simulink model "skarab_fgbe"  (R2018a)
settings: Solver=VariableStepDiscrete  StartTime=0.0  StopTime=50000  RelTol=1e-3
libraries: xbsIndex_r4 x704, casper_library_misc x5, xps_library x3
(part 3 of 9)

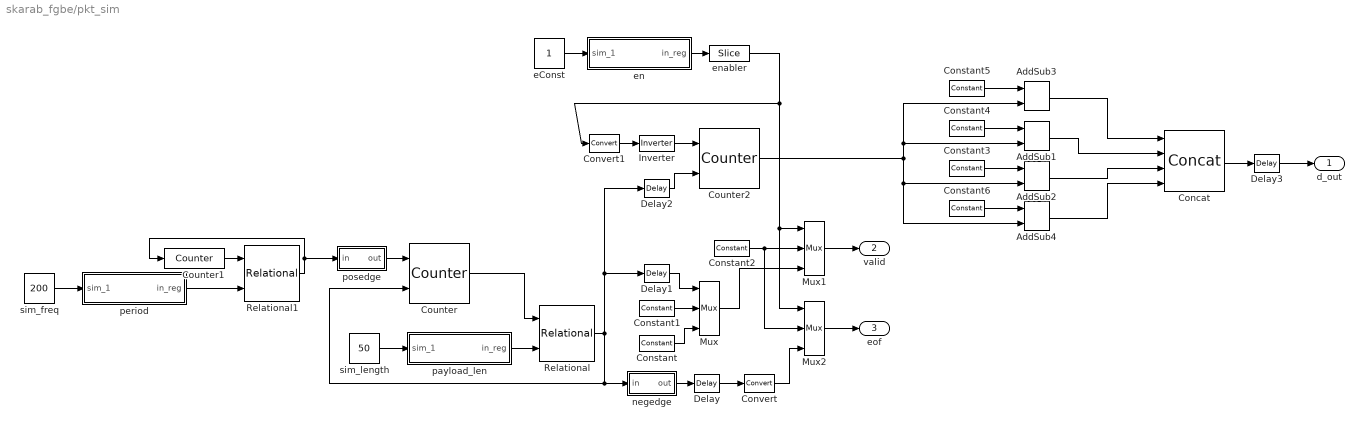
== system skarab_fgbe/pkt_sim ==
  AddSub{1..4} (4 alike) : xbsIndex_r4/AddSub  mode=Addition  use_carryin=off  use_carryout=off  en=off  latency=1  precision=User Defined  arith_type=Unsigned  n_bits=64  bin_pt=0  quantization=Truncate  overflow=Wrap  use_behavioral_HDL=off  hw_selection=Fabric  pipelined=off  dbl_ovrd=off  block_type=addsub
  Concat : xbsIndex_r4/Concat  num_inputs=4  dbl_ovrd=off  block_type=concat
  Constant : xbsIndex_r4/Constant  const=1  gui_display_data_type=Fixed-point  arith_type=Boolean  n_bits=16  bin_pt=14  preci_type=Single  exp_width=8  frac_width=24  explicit_period=on  period=1  equ=P=C  opselect=C  inp2=PCIN>>17  opr=+  inp1=P  carry=CIN  dbl_ovrd=off  block_type=constant
      settings: block_version=11.4
  Constant1 : xbsIndex_r4/Constant  const=0  gui_display_data_type=Fixed-point  arith_type=Boolean  n_bits=16  bin_pt=14  preci_type=Single  exp_width=8  frac_width=24  explicit_period=on  period=1  equ=P=C  opselect=C  inp2=PCIN>>17  opr=+  inp1=P  carry=CIN  dbl_ovrd=off  block_type=constant
      settings: block_version=11.4
  Constant2 : xbsIndex_r4/Constant  const=0  gui_display_data_type=Fixed-point  arith_type=Boolean  n_bits=16  bin_pt=14  preci_type=Single  exp_width=8  frac_width=24  explicit_period=on  period=1  equ=P=C  opselect=C  inp2=PCIN>>17  opr=+  inp1=P  carry=CIN  dbl_ovrd=off  block_type=constant
      settings: block_version=11.4
  Constant3 : xbsIndex_r4/Constant  const=3  gui_display_data_type=Fixed-point  arith_type=Unsigned  n_bits=64  bin_pt=0  preci_type=Single  exp_width=8  frac_width=24  explicit_period=off  period=1  equ=P=C  opselect=C  inp2=PCIN>>17  opr=+  inp1=P  carry=CIN  dbl_ovrd=off  block_type=constant
  Constant4 : xbsIndex_r4/Constant  const=2  gui_display_data_type=Fixed-point  arith_type=Unsigned  n_bits=64  bin_pt=0  preci_type=Single  exp_width=8  frac_width=24  explicit_period=off  period=1  equ=P=C  opselect=C  inp2=PCIN>>17  opr=+  inp1=P  carry=CIN  dbl_ovrd=off  block_type=constant
  Constant5 : xbsIndex_r4/Constant  const=1  gui_display_data_type=Fixed-point  arith_type=Unsigned  n_bits=64  bin_pt=0  preci_type=Single  exp_width=8  frac_width=24  explicit_period=off  period=1  equ=P=C  opselect=C  inp2=PCIN>>17  opr=+  inp1=P  carry=CIN  dbl_ovrd=off  block_type=constant
  Constant6 : xbsIndex_r4/Constant  const=4  gui_display_data_type=Fixed-point  arith_type=Unsigned  n_bits=64  bin_pt=0  preci_type=Single  exp_width=8  frac_width=24  explicit_period=off  period=1  equ=P=C  opselect=C  inp2=PCIN>>17  opr=+  inp1=P  carry=CIN  dbl_ovrd=off  block_type=constant
  Convert : xbsIndex_r4/Convert  gui_display_data_type=Fixed-point  arith_type=Boolean  n_bits=16  bin_pt=14  float_type=Single  exp_bits=8  fraction_bits=24  quantization=Truncate  overflow=Wrap  en=off  latency=0  pipeline=off  dbl_ovrd=off  block_type=convert
      settings: block_version=11.4
  Convert1 : xbsIndex_r4/Convert  gui_display_data_type=Fixed-point  arith_type=Boolean  n_bits=16  bin_pt=14  float_type=Single  exp_bits=8  fraction_bits=24  quantization=Truncate  overflow=Wrap  en=off  latency=0  pipeline=off  dbl_ovrd=off  block_type=convert
      settings: block_version=11.4
  Counter : xbsIndex_r4/Counter  cnt_type=Free Running  cnt_to=Inf  operation=Up  start_count=0  cnt_by_val=1  arith_type=Unsigned  n_bits=32  bin_pt=0  load_pin=off  rst=on  en=on  explicit_period=on  period=1  use_behavioral_HDL=off  implementation=Fabric  dbl_ovrd=off  block_type=counter
      settings: block_version=11.4
  Counter1 : xbsIndex_r4/Counter  cnt_type=Free Running  cnt_to=Inf  operation=Up  start_count=1  cnt_by_val=1  arith_type=Unsigned  n_bits=32  bin_pt=0  load_pin=off  rst=on  en=off  explicit_period=on  period=1  use_behavioral_HDL=off  implementation=Fabric  dbl_ovrd=off  block_type=counter
      settings: block_version=11.4
  Counter2 : xbsIndex_r4/Counter  cnt_type=Free Running  cnt_to=Inf  operation=Up  start_count=0  cnt_by_val=1  arith_type=Unsigned  n_bits=64  bin_pt=0  load_pin=off  rst=on  en=on  explicit_period=off  period=1  use_behavioral_HDL=off  implementation=Fabric  dbl_ovrd=off  block_type=counter
      settings: block_version=11.4
  Delay{,1..3} (4 alike) : xbsIndex_r4/Delay  rst=off  infoeditControl=Selection of Reset will increase slice count due to use of real FFs and instead of SRLs  en=off  latency=1  reg_retiming=on  dbl_ovrd=off  block_type=delay
      settings: block_version=11.4
  Inverter : xbsIndex_r4/Inverter  en=off  latency=0  dbl_ovrd=off  block_type=inv
      settings: block_version=11.4
  Mux : xbsIndex_r4/Mux  inputs=2  en=off  latency=1  precision=Full  arith_type=Unsigned  n_bits=16  bin_pt=14  quantization=Truncate  overflow=Wrap  dbl_ovrd=off  block_type=mux
      settings: block_version=11.4
  Mux1 : xbsIndex_r4/Mux  inputs=2  en=off  latency=1  precision=Full  arith_type=Unsigned  n_bits=16  bin_pt=14  quantization=Truncate  overflow=Wrap  dbl_ovrd=off  block_type=mux
      settings: block_version=11.4
  Mux2 : xbsIndex_r4/Mux  inputs=2  en=off  latency=1  precision=Full  arith_type=Unsigned  n_bits=16  bin_pt=14  quantization=Truncate  overflow=Wrap  dbl_ovrd=off  block_type=mux
      settings: block_version=11.4
  Relational : xbsIndex_r4/Relational  mode=a<b  op_type=Bool  en=off  latency=0  dbl_ovrd=off  block_type=relational
  Relational1 : xbsIndex_r4/Relational  mode=a>=b  op_type=Bool  en=off  latency=0  dbl_ovrd=off  block_type=relational
  eConst : Constant
  en : Subsystem  Tag=xps:sw_reg  AncestorBlock=xps_library/Memory/software_register  mask(swreg){io_dir=From Processor, io_delay=0, init_val=234000, sample_period=1, names=reg, bitwidths=32, bin_pts=0, arith_types=0, sim_port=on, show_format=on}
      mask prompts: io_dir "I/O direction"; io_delay "I/O delay"; init_val "Initial Value"; sample_period "Sample period"; names "Bitfield names [msb...lsb]"; bitwidths "Bitfield widths"; bin_pts "Bitfield binary pts"; arith_types "Bitfield types, ufix=0, fix=1, bool=2"; sim_port "Provide sim input/output?"; show_format "Print format string?"
      mask help: A 32-bit software-accessible register. Can be divided into bitfields of varying widths and types using the fields in the block mask.
      mask init:
      | swreg_init(gcb)
      settings: AttributesFormatString=1input:uf32.0 = 32 bits
      mask TypeOptions io_dir: To Processor | From Processor
      mask Callback io_dir:
      | mask_enables = get_param(gcb, 'MaskEnables');
      | mask_names = get_param(gcb, 'MaskNames');
      | if strcmp(get_param(gcb, 'io_dir'), 'To Processor'),
      |     mask_enables{ismember(mask_names, 'sample_period')} = 'off';
      | else
      |     mask_enables{ismember(mask_names, 'sample_period')} = 'on';
      | end
      | set_param(gcb, 'MaskEnables', mask_enables);
      mask DialogControl ParameterTabVar0 Prompt: Setup
  enabler : xbsIndex_r4/Slice  nbits=1  boolean_output=off  mode=Lower Bit Location + Width  bit1=0  base1=MSB of Input  bit0=0  base0=LSB of Input  dbl_ovrd=off  block_type=slice
  negedge : Subsystem  AncestorBlock=casper_library_misc/edge_detect  mask(edge_detect){edge=Falling, polarity=Active High, x_in=[0 0.08 0.08 0.16 0.16 0.24 0.24 0.32 0.32 0.4], y_in=[-1 -1  1  1  1  1  1  1  1  1], x_out=[0.6 0.68 0.68 0.76 0.76 0.84 0.84 0.92 0.92 1], y_out=[-1 -1  1  1 -1 -1 -1 -1 -1 -1]}
      mask prompts: edge "Edge Type"; polarity "Output Polarity"; x_in "Input X Positions"; y_in "Input Y Positions"; x_out "Output X Positions"; y_out "Output Y Positions"
      mask help: Output is active for one-cycle after each edge of the specified type (i.e. rising, falling or both).
      mask init:
      | edge_detect_init(gcb,...
      |     'edge',edge,...
      |     'polarity',polarity,...
      |     'x_in',x_in,...
      |     'x_out',x_out,...
      |     'y_in',y_in,...
      |     'y_out',y_out);
      | 
      | x_in_num=str2num(getfield(getfield(get_param(gcb,'UserData'),'parameters'),'x_in'));
      | x_out_num=str2num(getfield(getfield(get_param(gcb,'UserData'),'parameters'),'x_out'));
      | y_in_num=str2num(getfield(getfield(get_param(gcb,'UserData'),'parameters'),'y_in'));
      | y_out_num=str2num(getfield(getfield(get_param(gcb,'UserData'),'parameters'),'y_out'));
      settings: AttributesFormatString=|
      | falling edges
      | active high
      mask Help: Output is active for one-cycle after each edge of the specified type (i.e. rising, falling, or both).  Latency is zero.
      mask TypeOptions edge: Rising | Falling | Both
      mask TypeOptions polarity: Active High | Active Low
      mask Display:
      | plot(x_in_num,0.5+y_in_num*0.2);
      | plot(x_out_num,0.5+y_out_num*0.2);
  payload_len : Subsystem  Tag=xps:sw_reg  AncestorBlock=xps_library/Memory/software_register  mask(swreg){io_dir=From Processor, io_delay=0, init_val=654, sample_period=1, names=reg, bitwidths=32, bin_pts=0, arith_types=0, sim_port=on, show_format=on}
      mask prompts: io_dir "I/O direction"; io_delay "I/O delay"; init_val "Initial Value"; sample_period "Sample period"; names "Bitfield names [msb...lsb]"; bitwidths "Bitfield widths"; bin_pts "Bitfield binary pts"; arith_types "Bitfield types, ufix=0, fix=1, bool=2"; sim_port "Provide sim input/output?"; show_format "Print format string?"
      mask help: A 32-bit software-accessible register. Can be divided into bitfields of varying widths and types using the fields in the block mask.
      mask init:
      | swreg_init(gcb)
      settings: AttributesFormatString=1input:uf32.0 = 32 bits
      mask TypeOptions io_dir: To Processor | From Processor
      mask Callback io_dir:
      | mask_enables = get_param(gcb, 'MaskEnables');
      | mask_names = get_param(gcb, 'MaskNames');
      | if strcmp(get_param(gcb, 'io_dir'), 'To Processor'),
      |     mask_enables{ismember(mask_names, 'sample_period')} = 'off';
      | else
      |     mask_enables{ismember(mask_names, 'sample_period')} = 'on';
      | end
      | set_param(gcb, 'MaskEnables', mask_enables);
      mask DialogControl ParameterTabVar0 Prompt: Setup
  period : Subsystem  Tag=xps:sw_reg  AncestorBlock=xps_library/Memory/software_register  mask(swreg){io_dir=From Processor, io_delay=0, init_val=1000, sample_period=1, names=reg, bitwidths=32, bin_pts=0, arith_types=0, sim_port=on, show_format=on}
      mask prompts: io_dir "I/O direction"; io_delay "I/O delay"; init_val "Initial Value"; sample_period "Sample period"; names "Bitfield names [msb...lsb]"; bitwidths "Bitfield widths"; bin_pts "Bitfield binary pts"; arith_types "Bitfield types, ufix=0, fix=1, bool=2"; sim_port "Provide sim input/output?"; show_format "Print format string?"
      mask help: A 32-bit software-accessible register. Can be divided into bitfields of varying widths and types using the fields in the block mask.
      mask init:
      | swreg_init(gcb)
      settings: AttributesFormatString=1input:uf32.0 = 32 bits
      mask TypeOptions io_dir: To Processor | From Processor
      mask Callback io_dir:
      | mask_enables = get_param(gcb, 'MaskEnables');
      | mask_names = get_param(gcb, 'MaskNames');
      | if strcmp(get_param(gcb, 'io_dir'), 'To Processor'),
      |     mask_enables{ismember(mask_names, 'sample_period')} = 'off';
      | else
      |     mask_enables{ismember(mask_names, 'sample_period')} = 'on';
      | end
      | set_param(gcb, 'MaskEnables', mask_enables);
      mask DialogControl ParameterTabVar0 Prompt: Setup
  posedge : Subsystem  AncestorBlock=casper_library_misc/edge_detect  mask(edge_detect){edge=Rising, polarity=Active High, x_in=[0 0.08 0.08 0.16 0.16 0.24 0.24 0.32 0.32 0.4], y_in=[-1 -1  1  1  1  1  1  1  1  1], x_out=[0.6 0.68 0.68 0.76 0.76 0.84 0.84 0.92 0.92 1], y_out=[-1 -1  1  1 -1 -1 -1 -1 -1 -1]}
      mask prompts: edge "Edge Type"; polarity "Output Polarity"; x_in "Input X Positions"; y_in "Input Y Positions"; x_out "Output X Positions"; y_out "Output Y Positions"
      mask help: Output is active for one-cycle after each edge of the specified type (i.e. rising, falling or both).
      mask init: same as skarab_fgbe/pkt_sim/negedge
      settings: AttributesFormatString=|
      | rising edges
      | active high
      mask Help: Output is active for one-cycle after each edge of the specified type (i.e. rising, falling, or both).  Latency is zero.
      mask TypeOptions edge: Rising | Falling | Both
      mask TypeOptions polarity: Active High | Active Low
      mask Display:
      | plot(x_in_num,0.5+y_in_num*0.2);
      | plot(x_out_num,0.5+y_out_num*0.2);
  sim_freq : Constant  Value=200
  sim_length : Constant  Value=50
  d_out : Outport
  valid : Outport  Port=2
  eof : Outport  Port=3
  wires:
  Counter/1 -> Relational/1
  sim_length/1 -> payload_len/1(sim_1)
  posedge/1(out) -> Counter/1
  Mux2/1 -> eof/1
  Mux1/1 -> valid/1
  Delay3/1 -> d_out/1
  enabler/1 -> Mux1/1, Mux2/1, Convert1/1
  en/1(in_reg) -> enabler/1
  eConst/1 -> en/1(sim_1)
  Convert1/1 -> Inverter/1
  Inverter/1 -> Counter2/1
  Delay2/1 -> Counter2/2
  Convert/1 -> Mux2/3
  Constant2/1 -> Mux1/2, Mux2/2
  Mux/1 -> Mux1/3
  Delay1/1 -> Mux/1
  Constant/1 -> Mux/3
  Constant1/1 -> Mux/2
  Delay/1 -> Convert/1
  negedge/1(out) -> Delay/1
  Relational1/1 -> posedge/1(in), Counter1/1
  Counter1/1 -> Relational1/1
  period/1(in_reg) -> Relational1/2
  sim_freq/1 -> period/1(sim_1)
  Relational/1 -> negedge/1(in), Counter/2, Delay1/1, Delay2/1
  payload_len/1(in_reg) -> Relational/2
  Constant5/1 -> AddSub3/1
  Constant4/1 -> AddSub1/1
  Constant3/1 -> AddSub2/1
  Constant6/1 -> AddSub4/1
  Counter2/1 -> AddSub1/2, AddSub3/2, AddSub2/2, AddSub4/2
  AddSub3/1 -> Concat/1
  AddSub1/1 -> Concat/2
  AddSub2/1 -> Concat/3
  AddSub4/1 -> Concat/4
  Concat/1 -> Delay3/1

== system skarab_fgbe/rst ==
  sim_1 : Inport
  convert1_1 : DataTypeConversion  OutDataTypeStr=fixdt('ufix32_En0')  LockScale=on
  convert2_1 : DataTypeConversion  OutDataTypeStr=fixdt('ufix32_En0')  ConvertRealWorld=Stored Integer (SI)  LockScale=on
  gain_1 : Gain
  io_delay : xbsIndex_r4/Delay  rst=off  infoeditControl=Selection of Reset will increase slice count due to use of real FFs and instead of SRLs  en=off  latency=0  reg_retiming=on  dbl_ovrd=off  block_type=delay
  reint1 : xbsIndex_r4/Reinterpret  force_arith_type=on  arith_type=Unsigned  force_bin_pt=on  bin_pt=0  block_type=reinterpret
  skarab_fgbe_rst_user_data_out : xbsIndex_r4/Gateway In  gui_display_data_type=Fixed-point  arith_type=Unsigned  n_bits=32  bin_pt=0  preci_type=Single  exp_width=8  frac_width=24  rows=1  columns=1  quantization="Round  (unbiased: +/- Inf)"  overflow=Saturate  period=1  UseAsADC=off  ADCChannel='1'  interface=None  automatic_assignment=on  address_offset=hex2dec('00')  intf_name=''  intf_description=''  default_value=0  timing_constraint=None  locs_specified=off  LOCs={}  io_standard={}  inherit_from_input=off  hdl_port=on  dbl_ovrd=off  block_type=gatewayin
  slice_reg : xbsIndex_r4/Slice  nbits=32  boolean_output=off  mode=Lower Bit Location + Width  bit1=0  base1=MSB of Input  bit0=0  base0=LSB of Input  dbl_ovrd=off  block_type=slice
  in_reg : Outport
  wires:
  skarab_fgbe_rst_user_data_out/1 -> io_delay/1
  sim_1/1 -> convert1_1/1
  convert1_1/1 -> convert2_1/1
  convert2_1/1 -> gain_1/1
  gain_1/1 -> skarab_fgbe_rst_user_data_out/1
  io_delay/1 -> slice_reg/1
  slice_reg/1 -> reint1/1
  reint1/1 -> in_reg/1

== system skarab_fgbe/rx ==
  out_reg : Inport
  assert_reg : xbsIndex_r4/Assert  assert_type=on  type_source=Explicitly  gui_display_data_type=Fixed-point  arith_type=Unsigned  n_bits=32  bin_pt=0  preci_type=Single  exp_width=8  frac_width=24  assert_rate=off  rate_source=Explicitly  period=1  output_port=on  block_type=assert
  cast_gw : xbsIndex_r4/Convert  gui_display_data_type=Fixed-point  arith_type=Unsigned  n_bits=32  bin_pt=0  float_type=Single  exp_bits=8  fraction_bits=24  quantization=Truncate  overflow=Wrap  en=off  latency=1  pipeline=off  dbl_ovrd=off  block_type=convert
  io_delay : xbsIndex_r4/Delay  rst=off  infoeditControl=Selection of Reset will increase slice count due to use of real FFs and instead of SRLs  en=off  latency=0  reg_retiming=on  dbl_ovrd=off  block_type=delay
  reint1 : xbsIndex_r4/Reinterpret  force_arith_type=on  arith_type=Unsigned  force_bin_pt=on  bin_pt=0  block_type=reinterpret
  sim_out : Terminator
  sim_out_reg_gw : xbsIndex_r4/Gateway Out  inherit_from_input=off  hdl_port=off  rows=1  columns=1  UseAsDAC=off  DACChannel='1'  interface=None  automatic_assignment=on  address_offset=hex2dec('00')  intf_name=''  intf_description=''  timing_constraint=None  locs_specified=off  LOCs={}  io_standard={}  block_type=gatewayout
  sim_out_reg_sim_delay : xbsIndex_r4/Delay  rst=off  infoeditControl=Selection of Reset will increase slice count due to use of real FFs and instead of SRLs  en=off  latency=1  reg_retiming=on  dbl_ovrd=off  block_type=delay
  skarab_fgbe_rx_user_data_in : xbsIndex_r4/Gateway Out  inherit_from_input=off  hdl_port=on  rows=1  columns=1  UseAsDAC=off  DACChannel='1'  interface=None  automatic_assignment=on  address_offset=hex2dec('00')  intf_name=''  intf_description=''  timing_constraint=None  locs_specified=off  LOCs={}  io_standard={}  block_type=gatewayout
  sim_out_reg : Outport
  wires:
  sim_out_reg_sim_delay/1 -> sim_out_reg_gw/1
  sim_out_reg_gw/1 -> sim_out_reg/1
  io_delay/1 -> cast_gw/1
  cast_gw/1 -> skarab_fgbe_rx_user_data_in/1
  skarab_fgbe_rx_user_data_in/1 -> sim_out/1
  out_reg/1 -> sim_out_reg_sim_delay/1, assert_reg/1
  assert_reg/1 -> reint1/1
  reint1/1 -> io_delay/1

== system skarab_fgbe/rx_bad_frame ==
  out_reg : Inport
  assert_reg : xbsIndex_r4/Assert  assert_type=on  type_source=Explicitly  gui_display_data_type=Fixed-point  arith_type=Unsigned  n_bits=32  bin_pt=0  preci_type=Single  exp_width=8  frac_width=24  assert_rate=off  rate_source=Explicitly  period=1  output_port=on  block_type=assert
  cast_gw : xbsIndex_r4/Convert  gui_display_data_type=Fixed-point  arith_type=Unsigned  n_bits=32  bin_pt=0  float_type=Single  exp_bits=8  fraction_bits=24  quantization=Truncate  overflow=Wrap  en=off  latency=1  pipeline=off  dbl_ovrd=off  block_type=convert
  io_delay : xbsIndex_r4/Delay  rst=off  infoeditControl=Selection of Reset will increase slice count due to use of real FFs and instead of SRLs  en=off  latency=0  reg_retiming=on  dbl_ovrd=off  block_type=delay
  reint1 : xbsIndex_r4/Reinterpret  force_arith_type=on  arith_type=Unsigned  force_bin_pt=on  bin_pt=0  block_type=reinterpret
  sim_out : Terminator
  sim_out_reg_gw : xbsIndex_r4/Gateway Out  inherit_from_input=off  hdl_port=off  rows=1  columns=1  UseAsDAC=off  DACChannel='1'  interface=None  automatic_assignment=on  address_offset=hex2dec('00')  intf_name=''  intf_description=''  timing_constraint=None  locs_specified=off  LOCs={}  io_standard={}  block_type=gatewayout
  sim_out_reg_sim_delay : xbsIndex_r4/Delay  rst=off  infoeditControl=Selection of Reset will increase slice count due to use of real FFs and instead of SRLs  en=off  latency=1  reg_retiming=on  dbl_ovrd=off  block_type=delay
  skarab_fgbe_rx_bad_frame_user_data_in : xbsIndex_r4/Gateway Out  inherit_from_input=off  hdl_port=on  rows=1  columns=1  UseAsDAC=off  DACChannel='1'  interface=None  automatic_assignment=on  address_offset=hex2dec('00')  intf_name=''  intf_description=''  timing_constraint=None  locs_specified=off  LOCs={}  io_standard={}  block_type=gatewayout
  sim_out_reg : Outport
  wires:
  sim_out_reg_sim_delay/1 -> sim_out_reg_gw/1
  sim_out_reg_gw/1 -> sim_out_reg/1
  io_delay/1 -> cast_gw/1
  cast_gw/1 -> skarab_fgbe_rx_bad_frame_user_data_in/1
  skarab_fgbe_rx_bad_frame_user_data_in/1 -> sim_out/1
  out_reg/1 -> sim_out_reg_sim_delay/1, assert_reg/1
  assert_reg/1 -> reint1/1
  reint1/1 -> io_delay/1

== system skarab_fgbe/rx_data ==
  out_reg : Inport
  assert_reg : xbsIndex_r4/Assert  assert_type=on  type_source=Explicitly  gui_display_data_type=Fixed-point  arith_type=Unsigned  n_bits=32  bin_pt=0  preci_type=Single  exp_width=8  frac_width=24  assert_rate=off  rate_source=Explicitly  period=1  output_port=on  block_type=assert
  cast_gw : xbsIndex_r4/Convert  gui_display_data_type=Fixed-point  arith_type=Unsigned  n_bits=32  bin_pt=0  float_type=Single  exp_bits=8  fraction_bits=24  quantization=Truncate  overflow=Wrap  en=off  latency=1  pipeline=off  dbl_ovrd=off  block_type=convert
  io_delay : xbsIndex_r4/Delay  rst=off  infoeditControl=Selection of Reset will increase slice count due to use of real FFs and instead of SRLs  en=off  latency=0  reg_retiming=on  dbl_ovrd=off  block_type=delay
  reint1 : xbsIndex_r4/Reinterpret  force_arith_type=on  arith_type=Unsigned  force_bin_pt=on  bin_pt=0  block_type=reinterpret
  sim_out : Terminator
  sim_out_reg_gw : xbsIndex_r4/Gateway Out  inherit_from_input=off  hdl_port=off  rows=1  columns=1  UseAsDAC=off  DACChannel='1'  interface=None  automatic_assignment=on  address_offset=hex2dec('00')  intf_name=''  intf_description=''  timing_constraint=None  locs_specified=off  LOCs={}  io_standard={}  block_type=gatewayout
  sim_out_reg_sim_delay : xbsIndex_r4/Delay  rst=off  infoeditControl=Selection of Reset will increase slice count due to use of real FFs and instead of SRLs  en=off  latency=1  reg_retiming=on  dbl_ovrd=off  block_type=delay
  skarab_fgbe_rx_data_user_data_in : xbsIndex_r4/Gateway Out  inherit_from_input=off  hdl_port=on  rows=1  columns=1  UseAsDAC=off  DACChannel='1'  interface=None  automatic_assignment=on  address_offset=hex2dec('00')  intf_name=''  intf_description=''  timing_constraint=None  locs_specified=off  LOCs={}  io_standard={}  block_type=gatewayout
  sim_out_reg : Outport
  wires:
  sim_out_reg_sim_delay/1 -> sim_out_reg_gw/1
  sim_out_reg_gw/1 -> sim_out_reg/1
  io_delay/1 -> cast_gw/1
  cast_gw/1 -> skarab_fgbe_rx_data_user_data_in/1
  skarab_fgbe_rx_data_user_data_in/1 -> sim_out/1
  out_reg/1 -> sim_out_reg_sim_delay/1, assert_reg/1
  assert_reg/1 -> reint1/1
  reint1/1 -> io_delay/1

== system skarab_fgbe/rx_dest_ip ==
  out_reg : Inport
  assert_reg : xbsIndex_r4/Assert  assert_type=on  type_source=Explicitly  gui_display_data_type=Fixed-point  arith_type=Unsigned  n_bits=32  bin_pt=0  preci_type=Single  exp_width=8  frac_width=24  assert_rate=off  rate_source=Explicitly  period=1  output_port=on  block_type=assert
  cast_gw : xbsIndex_r4/Convert  gui_display_data_type=Fixed-point  arith_type=Unsigned  n_bits=32  bin_pt=0  float_type=Single  exp_bits=8  fraction_bits=24  quantization=Truncate  overflow=Wrap  en=off  latency=1  pipeline=off  dbl_ovrd=off  block_type=convert
  io_delay : xbsIndex_r4/Delay  rst=off  infoeditControl=Selection of Reset will increase slice count due to use of real FFs and instead of SRLs  en=off  latency=0  reg_retiming=on  dbl_ovrd=off  block_type=delay
  reint1 : xbsIndex_r4/Reinterpret  force_arith_type=on  arith_type=Unsigned  force_bin_pt=on  bin_pt=0  block_type=reinterpret
  sim_out : Terminator
  sim_out_reg_gw : xbsIndex_r4/Gateway Out  inherit_from_input=off  hdl_port=off  rows=1  columns=1  UseAsDAC=off  DACChannel='1'  interface=None  automatic_assignment=on  address_offset=hex2dec('00')  intf_name=''  intf_description=''  timing_constraint=None  locs_specified=off  LOCs={}  io_standard={}  block_type=gatewayout
  sim_out_reg_sim_delay : xbsIndex_r4/Delay  rst=off  infoeditControl=Selection of Reset will increase slice count due to use of real FFs and instead of SRLs  en=off  latency=1  reg_retiming=on  dbl_ovrd=off  block_type=delay
  skarab_fgbe_rx_dest_ip_user_data_in : xbsIndex_r4/Gateway Out  inherit_from_input=off  hdl_port=on  rows=1  columns=1  UseAsDAC=off  DACChannel='1'  interface=None  automatic_assignment=on  address_offset=hex2dec('00')  intf_name=''  intf_description=''  timing_constraint=None  locs_specified=off  LOCs={}  io_standard={}  block_type=gatewayout
  sim_out_reg : Outport
  wires:
  sim_out_reg_sim_delay/1 -> sim_out_reg_gw/1
  sim_out_reg_gw/1 -> sim_out_reg/1
  io_delay/1 -> cast_gw/1
  cast_gw/1 -> skarab_fgbe_rx_dest_ip_user_data_in/1
  skarab_fgbe_rx_dest_ip_user_data_in/1 -> sim_out/1
  out_reg/1 -> sim_out_reg_sim_delay/1, assert_reg/1
  assert_reg/1 -> reint1/1
  reint1/1 -> io_delay/1

== system skarab_fgbe/rx_dest_port ==
  out_reg : Inport
  assert_reg : xbsIndex_r4/Assert  assert_type=on  type_source=Explicitly  gui_display_data_type=Fixed-point  arith_type=Unsigned  n_bits=32  bin_pt=0  preci_type=Single  exp_width=8  frac_width=24  assert_rate=off  rate_source=Explicitly  period=1  output_port=on  block_type=assert
  cast_gw : xbsIndex_r4/Convert  gui_display_data_type=Fixed-point  arith_type=Unsigned  n_bits=32  bin_pt=0  float_type=Single  exp_bits=8  fraction_bits=24  quantization=Truncate  overflow=Wrap  en=off  latency=1  pipeline=off  dbl_ovrd=off  block_type=convert
  io_delay : xbsIndex_r4/Delay  rst=off  infoeditControl=Selection of Reset will increase slice count due to use of real FFs and instead of SRLs  en=off  latency=0  reg_retiming=on  dbl_ovrd=off  block_type=delay
  reint1 : xbsIndex_r4/Reinterpret  force_arith_type=on  arith_type=Unsigned  force_bin_pt=on  bin_pt=0  block_type=reinterpret
  sim_out : Terminator
  sim_out_reg_gw : xbsIndex_r4/Gateway Out  inherit_from_input=off  hdl_port=off  rows=1  columns=1  UseAsDAC=off  DACChannel='1'  interface=None  automatic_assignment=on  address_offset=hex2dec('00')  intf_name=''  intf_description=''  timing_constraint=None  locs_specified=off  LOCs={}  io_standard={}  block_type=gatewayout
  sim_out_reg_sim_delay : xbsIndex_r4/Delay  rst=off  infoeditControl=Selection of Reset will increase slice count due to use of real FFs and instead of SRLs  en=off  latency=1  reg_retiming=on  dbl_ovrd=off  block_type=delay
  skarab_fgbe_rx_dest_port_user_data_in : xbsIndex_r4/Gateway Out  inherit_from_input=off  hdl_port=on  rows=1  columns=1  UseAsDAC=off  DACChannel='1'  interface=None  automatic_assignment=on  address_offset=hex2dec('00')  intf_name=''  intf_description=''  timing_constraint=None  locs_specified=off  LOCs={}  io_standard={}  block_type=gatewayout
  sim_out_reg : Outport
  wires:
  sim_out_reg_sim_delay/1 -> sim_out_reg_gw/1
  sim_out_reg_gw/1 -> sim_out_reg/1
  io_delay/1 -> cast_gw/1
  cast_gw/1 -> skarab_fgbe_rx_dest_port_user_data_in/1
  skarab_fgbe_rx_dest_port_user_data_in/1 -> sim_out/1
  out_reg/1 -> sim_out_reg_sim_delay/1, assert_reg/1
  assert_reg/1 -> reint1/1
  reint1/1 -> io_delay/1

== system skarab_fgbe/rx_end_of_frame ==
  out_reg : Inport
  assert_reg : xbsIndex_r4/Assert  assert_type=on  type_source=Explicitly  gui_display_data_type=Fixed-point  arith_type=Unsigned  n_bits=32  bin_pt=0  preci_type=Single  exp_width=8  frac_width=24  assert_rate=off  rate_source=Explicitly  period=1  output_port=on  block_type=assert
  cast_gw : xbsIndex_r4/Convert  gui_display_data_type=Fixed-point  arith_type=Unsigned  n_bits=32  bin_pt=0  float_type=Single  exp_bits=8  fraction_bits=24  quantization=Truncate  overflow=Wrap  en=off  latency=1  pipeline=off  dbl_ovrd=off  block_type=convert
  io_delay : xbsIndex_r4/Delay  rst=off  infoeditControl=Selection of Reset will increase slice count due to use of real FFs and instead of SRLs  en=off  latency=0  reg_retiming=on  dbl_ovrd=off  block_type=delay
  reint1 : xbsIndex_r4/Reinterpret  force_arith_type=on  arith_type=Unsigned  force_bin_pt=on  bin_pt=0  block_type=reinterpret
  sim_out : Terminator
  sim_out_reg_gw : xbsIndex_r4/Gateway Out  inherit_from_input=off  hdl_port=off  rows=1  columns=1  UseAsDAC=off  DACChannel='1'  interface=None  automatic_assignment=on  address_offset=hex2dec('00')  intf_name=''  intf_description=''  timing_constraint=None  locs_specified=off  LOCs={}  io_standard={}  block_type=gatewayout
  sim_out_reg_sim_delay : xbsIndex_r4/Delay  rst=off  infoeditControl=Selection of Reset will increase slice count due to use of real FFs and instead of SRLs  en=off  latency=1  reg_retiming=on  dbl_ovrd=off  block_type=delay
  skarab_fgbe_rx_end_of_frame_user_data_in : xbsIndex_r4/Gateway Out  inherit_from_input=off  hdl_port=on  rows=1  columns=1  UseAsDAC=off  DACChannel='1'  interface=None  automatic_assignment=on  address_offset=hex2dec('00')  intf_name=''  intf_description=''  timing_constraint=None  locs_specified=off  LOCs={}  io_standard={}  block_type=gatewayout
  sim_out_reg : Outport
  wires:
  sim_out_reg_sim_delay/1 -> sim_out_reg_gw/1
  sim_out_reg_gw/1 -> sim_out_reg/1
  io_delay/1 -> cast_gw/1
  cast_gw/1 -> skarab_fgbe_rx_end_of_frame_user_data_in/1
  skarab_fgbe_rx_end_of_frame_user_data_in/1 -> sim_out/1
  out_reg/1 -> sim_out_reg_sim_delay/1, assert_reg/1
  assert_reg/1 -> reint1/1
  reint1/1 -> io_delay/1

== system skarab_fgbe/rx_valid ==
  out_reg : Inport
  assert_reg : xbsIndex_r4/Assert  assert_type=on  type_source=Explicitly  gui_display_data_type=Fixed-point  arith_type=Unsigned  n_bits=32  bin_pt=0  preci_type=Single  exp_width=8  frac_width=24  assert_rate=off  rate_source=Explicitly  period=1  output_port=on  block_type=assert
  cast_gw : xbsIndex_r4/Convert  gui_display_data_type=Fixed-point  arith_type=Unsigned  n_bits=32  bin_pt=0  float_type=Single  exp_bits=8  fraction_bits=24  quantization=Truncate  overflow=Wrap  en=off  latency=1  pipeline=off  dbl_ovrd=off  block_type=convert
  io_delay : xbsIndex_r4/Delay  rst=off  infoeditControl=Selection of Reset will increase slice count due to use of real FFs and instead of SRLs  en=off  latency=0  reg_retiming=on  dbl_ovrd=off  block_type=delay
  reint1 : xbsIndex_r4/Reinterpret  force_arith_type=on  arith_type=Unsigned  force_bin_pt=on  bin_pt=0  block_type=reinterpret
  sim_out : Terminator
  sim_out_reg_gw : xbsIndex_r4/Gateway Out  inherit_from_input=off  hdl_port=off  rows=1  columns=1  UseAsDAC=off  DACChannel='1'  interface=None  automatic_assignment=on  address_offset=hex2dec('00')  intf_name=''  intf_description=''  timing_constraint=None  locs_specified=off  LOCs={}  io_standard={}  block_type=gatewayout
  sim_out_reg_sim_delay : xbsIndex_r4/Delay  rst=off  infoeditControl=Selection of Reset will increase slice count due to use of real FFs and instead of SRLs  en=off  latency=1  reg_retiming=on  dbl_ovrd=off  block_type=delay
  skarab_fgbe_rx_valid_user_data_in : xbsIndex_r4/Gateway Out  inherit_from_input=off  hdl_port=on  rows=1  columns=1  UseAsDAC=off  DACChannel='1'  interface=None  automatic_assignment=on  address_offset=hex2dec('00')  intf_name=''  intf_description=''  timing_constraint=None  locs_specified=off  LOCs={}  io_standard={}  block_type=gatewayout
  sim_out_reg : Outport
  wires:
  sim_out_reg_sim_delay/1 -> sim_out_reg_gw/1
  sim_out_reg_gw/1 -> sim_out_reg/1
  io_delay/1 -> cast_gw/1
  cast_gw/1 -> skarab_fgbe_rx_valid_user_data_in/1
  skarab_fgbe_rx_valid_user_data_in/1 -> sim_out/1
  out_reg/1 -> sim_out_reg_sim_delay/1, assert_reg/1
  assert_reg/1 -> reint1/1
  reint1/1 -> io_delay/1

== system skarab_fgbe/tx ==
  out_reg : Inport
  assert_reg : xbsIndex_r4/Assert  assert_type=on  type_source=Explicitly  gui_display_data_type=Fixed-point  arith_type=Unsigned  n_bits=32  bin_pt=0  preci_type=Single  exp_width=8  frac_width=24  assert_rate=off  rate_source=Explicitly  period=1  output_port=on  block_type=assert
  cast_gw : xbsIndex_r4/Convert  gui_display_data_type=Fixed-point  arith_type=Unsigned  n_bits=32  bin_pt=0  float_type=Single  exp_bits=8  fraction_bits=24  quantization=Truncate  overflow=Wrap  en=off  latency=1  pipeline=off  dbl_ovrd=off  block_type=convert
  io_delay : xbsIndex_r4/Delay  rst=off  infoeditControl=Selection of Reset will increase slice count due to use of real FFs and instead of SRLs  en=off  latency=0  reg_retiming=on  dbl_ovrd=off  block_type=delay
  reint1 : xbsIndex_r4/Reinterpret  force_arith_type=on  arith_type=Unsigned  force_bin_pt=on  bin_pt=0  block_type=reinterpret
  sim_out : Terminator
  sim_out_reg_gw : xbsIndex_r4/Gateway Out  inherit_from_input=off  hdl_port=off  rows=1  columns=1  UseAsDAC=off  DACChannel='1'  interface=None  automatic_assignment=on  address_offset=hex2dec('00')  intf_name=''  intf_description=''  timing_constraint=None  locs_specified=off  LOCs={}  io_standard={}  block_type=gatewayout
  sim_out_reg_sim_delay : xbsIndex_r4/Delay  rst=off  infoeditControl=Selection of Reset will increase slice count due to use of real FFs and instead of SRLs  en=off  latency=1  reg_retiming=on  dbl_ovrd=off  block_type=delay
  skarab_fgbe_tx_user_data_in : xbsIndex_r4/Gateway Out  inherit_from_input=off  hdl_port=on  rows=1  columns=1  UseAsDAC=off  DACChannel='1'  interface=None  automatic_assignment=on  address_offset=hex2dec('00')  intf_name=''  intf_description=''  timing_constraint=None  locs_specified=off  LOCs={}  io_standard={}  block_type=gatewayout
  sim_out_reg : Outport
  wires:
  sim_out_reg_sim_delay/1 -> sim_out_reg_gw/1
  sim_out_reg_gw/1 -> sim_out_reg/1
  io_delay/1 -> cast_gw/1
  cast_gw/1 -> skarab_fgbe_tx_user_data_in/1
  skarab_fgbe_tx_user_data_in/1 -> sim_out/1
  out_reg/1 -> sim_out_reg_sim_delay/1, assert_reg/1
  assert_reg/1 -> reint1/1
  reint1/1 -> io_delay/1

== system skarab_fgbe/tx_cnt ==
  out_reg : Inport
  assert_reg : xbsIndex_r4/Assert  assert_type=on  type_source=Explicitly  gui_display_data_type=Fixed-point  arith_type=Unsigned  n_bits=32  bin_pt=0  preci_type=Single  exp_width=8  frac_width=24  assert_rate=off  rate_source=Explicitly  period=1  output_port=on  block_type=assert
  cast_gw : xbsIndex_r4/Convert  gui_display_data_type=Fixed-point  arith_type=Unsigned  n_bits=32  bin_pt=0  float_type=Single  exp_bits=8  fraction_bits=24  quantization=Truncate  overflow=Wrap  en=off  latency=1  pipeline=off  dbl_ovrd=off  block_type=convert
  io_delay : xbsIndex_r4/Delay  rst=off  infoeditControl=Selection of Reset will increase slice count due to use of real FFs and instead of SRLs  en=off  latency=0  reg_retiming=on  dbl_ovrd=off  block_type=delay
  reint1 : xbsIndex_r4/Reinterpret  force_arith_type=on  arith_type=Unsigned  force_bin_pt=on  bin_pt=0  block_type=reinterpret
  sim_out : Terminator
  sim_out_reg_gw : xbsIndex_r4/Gateway Out  inherit_from_input=off  hdl_port=off  rows=1  columns=1  UseAsDAC=off  DACChannel='1'  interface=None  automatic_assignment=on  address_offset=hex2dec('00')  intf_name=''  intf_description=''  timing_constraint=None  locs_specified=off  LOCs={}  io_standard={}  block_type=gatewayout
  sim_out_reg_sim_delay : xbsIndex_r4/Delay  rst=off  infoeditControl=Selection of Reset will increase slice count due to use of real FFs and instead of SRLs  en=off  latency=1  reg_retiming=on  dbl_ovrd=off  block_type=delay
  skarab_fgbe_tx_cnt_user_data_in : xbsIndex_r4/Gateway Out  inherit_from_input=off  hdl_port=on  rows=1  columns=1  UseAsDAC=off  DACChannel='1'  interface=None  automatic_assignment=on  address_offset=hex2dec('00')  intf_name=''  intf_description=''  timing_constraint=None  locs_specified=off  LOCs={}  io_standard={}  block_type=gatewayout
  sim_out_reg : Outport
  wires:
  sim_out_reg_sim_delay/1 -> sim_out_reg_gw/1
  sim_out_reg_gw/1 -> sim_out_reg/1
  io_delay/1 -> cast_gw/1
  cast_gw/1 -> skarab_fgbe_tx_cnt_user_data_in/1
  skarab_fgbe_tx_cnt_user_data_in/1 -> sim_out/1
  out_reg/1 -> sim_out_reg_sim_delay/1, assert_reg/1
  assert_reg/1 -> reint1/1
  reint1/1 -> io_delay/1

== system skarab_fgbe/tx_full ==
  out_reg : Inport
  assert_reg : xbsIndex_r4/Assert  assert_type=on  type_source=Explicitly  gui_display_data_type=Fixed-point  arith_type=Unsigned  n_bits=32  bin_pt=0  preci_type=Single  exp_width=8  frac_width=24  assert_rate=off  rate_source=Explicitly  period=1  output_port=on  block_type=assert
  cast_gw : xbsIndex_r4/Convert  gui_display_data_type=Fixed-point  arith_type=Unsigned  n_bits=32  bin_pt=0  float_type=Single  exp_bits=8  fraction_bits=24  quantization=Truncate  overflow=Wrap  en=off  latency=1  pipeline=off  dbl_ovrd=off  block_type=convert
  io_delay : xbsIndex_r4/Delay  rst=off  infoeditControl=Selection of Reset will increase slice count due to use of real FFs and instead of SRLs  en=off  latency=0  reg_retiming=on  dbl_ovrd=off  block_type=delay
  reint1 : xbsIndex_r4/Reinterpret  force_arith_type=on  arith_type=Unsigned  force_bin_pt=on  bin_pt=0  block_type=reinterpret
  sim_out : Terminator
  sim_out_reg_gw : xbsIndex_r4/Gateway Out  inherit_from_input=off  hdl_port=off  rows=1  columns=1  UseAsDAC=off  DACChannel='1'  interface=None  automatic_assignment=on  address_offset=hex2dec('00')  intf_name=''  intf_description=''  timing_constraint=None  locs_specified=off  LOCs={}  io_standard={}  block_type=gatewayout
  sim_out_reg_sim_delay : xbsIndex_r4/Delay  rst=off  infoeditControl=Selection of Reset will increase slice count due to use of real FFs and instead of SRLs  en=off  latency=1  reg_retiming=on  dbl_ovrd=off  block_type=delay
  skarab_fgbe_tx_full_user_data_in : xbsIndex_r4/Gateway Out  inherit_from_input=off  hdl_port=on  rows=1  columns=1  UseAsDAC=off  DACChannel='1'  interface=None  automatic_assignment=on  address_offset=hex2dec('00')  intf_name=''  intf_description=''  timing_constraint=None  locs_specified=off  LOCs={}  io_standard={}  block_type=gatewayout
  sim_out_reg : Outport
  wires:
  sim_out_reg_sim_delay/1 -> sim_out_reg_gw/1
  sim_out_reg_gw/1 -> sim_out_reg/1
  io_delay/1 -> cast_gw/1
  cast_gw/1 -> skarab_fgbe_tx_full_user_data_in/1
  skarab_fgbe_tx_full_user_data_in/1 -> sim_out/1
  out_reg/1 -> sim_out_reg_sim_delay/1, assert_reg/1
  assert_reg/1 -> reint1/1
  reint1/1 -> io_delay/1

== system skarab_fgbe/tx_overflow ==
  out_reg : Inport
  assert_reg : xbsIndex_r4/Assert  assert_type=on  type_source=Explicitly  gui_display_data_type=Fixed-point  arith_type=Unsigned  n_bits=32  bin_pt=0  preci_type=Single  exp_width=8  frac_width=24  assert_rate=off  rate_source=Explicitly  period=1  output_port=on  block_type=assert
  cast_gw : xbsIndex_r4/Convert  gui_display_data_type=Fixed-point  arith_type=Unsigned  n_bits=32  bin_pt=0  float_type=Single  exp_bits=8  fraction_bits=24  quantization=Truncate  overflow=Wrap  en=off  latency=1  pipeline=off  dbl_ovrd=off  block_type=convert
  io_delay : xbsIndex_r4/Delay  rst=off  infoeditControl=Selection of Reset will increase slice count due to use of real FFs and instead of SRLs  en=off  latency=0  reg_retiming=on  dbl_ovrd=off  block_type=delay
  reint1 : xbsIndex_r4/Reinterpret  force_arith_type=on  arith_type=Unsigned  force_bin_pt=on  bin_pt=0  block_type=reinterpret
  sim_out : Terminator
  sim_out_reg_gw : xbsIndex_r4/Gateway Out  inherit_from_input=off  hdl_port=off  rows=1  columns=1  UseAsDAC=off  DACChannel='1'  interface=None  automatic_assignment=on  address_offset=hex2dec('00')  intf_name=''  intf_description=''  timing_constraint=None  locs_specified=off  LOCs={}  io_standard={}  block_type=gatewayout
  sim_out_reg_sim_delay : xbsIndex_r4/Delay  rst=off  infoeditControl=Selection of Reset will increase slice count due to use of real FFs and instead of SRLs  en=off  latency=1  reg_retiming=on  dbl_ovrd=off  block_type=delay
  skarab_fgbe_tx_overflow_user_data_in : xbsIndex_r4/Gateway Out  inherit_from_input=off  hdl_port=on  rows=1  columns=1  UseAsDAC=off  DACChannel='1'  interface=None  automatic_assignment=on  address_offset=hex2dec('00')  intf_name=''  intf_description=''  timing_constraint=None  locs_specified=off  LOCs={}  io_standard={}  block_type=gatewayout
  sim_out_reg : Outport
  wires:
  sim_out_reg_sim_delay/1 -> sim_out_reg_gw/1
  sim_out_reg_gw/1 -> sim_out_reg/1
  io_delay/1 -> cast_gw/1
  cast_gw/1 -> skarab_fgbe_tx_overflow_user_data_in/1
  skarab_fgbe_tx_overflow_user_data_in/1 -> sim_out/1
  out_reg/1 -> sim_out_reg_sim_delay/1, assert_reg/1
  assert_reg/1 -> reint1/1
  reint1/1 -> io_delay/1

== system skarab_fgbe/forty_gbe/convert_tx_valid ==
  in : Inport
  bussify : Subsystem  AncestorBlock=casper_library_flow_control/bus_create  mask(bus_create){inputNum=4}
      mask prompts: inputNum "Number of inputs:"
      mask init:
      | bus_create_init(gcb,...
      |     'inputNum', inputNum);
  out : Outport
  wires:
  in/1 -> bussify/1(in1), bussify/2(in2), bussify/3(in3), bussify/4(in4)
  bussify/1(bus_out) -> out/1

== system skarab_fgbe/forty_gbe/pipeline_led_rx ==
  d : Inport
  q : Outport
  wires:
  d/1 -> q/1

== system skarab_fgbe/forty_gbe/pipeline_led_tx ==
  d : Inport
  q : Outport
  wires:
  d/1 -> q/1

== system skarab_fgbe/forty_gbe/pipeline_led_up ==
  d : Inport
  q : Outport
  wires:
  d/1 -> q/1

== system skarab_fgbe/forty_gbe/pipeline_rx_bad_frame ==
  d : Inport
  q : Outport
  wires:
  d/1 -> q/1

== system skarab_fgbe/forty_gbe/pipeline_rx_data ==
  d : Inport
  q : Outport
  wires:
  d/1 -> q/1

== system skarab_fgbe/forty_gbe/pipeline_rx_dest_ip ==
  d : Inport
  q : Outport
  wires:
  d/1 -> q/1

== system skarab_fgbe/forty_gbe/pipeline_rx_dest_port ==
  d : Inport
  q : Outport
  wires:
  d/1 -> q/1

== system skarab_fgbe/forty_gbe/pipeline_rx_end_of_frame ==
  d : Inport
  q : Outport
  wires:
  d/1 -> q/1

== system skarab_fgbe/forty_gbe/pipeline_rx_overrun ==
  d : Inport
  q : Outport
  wires:
  d/1 -> q/1

== system skarab_fgbe/forty_gbe/pipeline_rx_source_ip ==
  d : Inport
  q : Outport
  wires:
  d/1 -> q/1

== system skarab_fgbe/forty_gbe/pipeline_rx_source_port ==
  d : Inport
  q : Outport
  wires:
  d/1 -> q/1

== system skarab_fgbe/forty_gbe/pipeline_rx_valid ==
  d : Inport
  q : Outport
  wires:
  d/1 -> q/1

== system skarab_fgbe/forty_gbe/pipeline_tx_afull ==
  d : Inport
  q : Outport
  wires:
  d/1 -> q/1

== system skarab_fgbe/forty_gbe/pipeline_tx_overflow ==
  d : Inport
  q : Outport
  wires:
  d/1 -> q/1

== system skarab_fgbe/forty_gbe/rx_dv_or_exp ==
  bus_in : Inport
  slice1 : xbsIndex_r4/Slice  nbits=1  boolean_output=on  mode=Upper Bit Location + Width  bit1=-3  base1=MSB of Input  bit0=0  base0=LSB of Input  dbl_ovrd=off  block_type=slice
  slice2 : xbsIndex_r4/Slice  nbits=1  boolean_output=on  mode=Upper Bit Location + Width  bit1=-2  base1=MSB of Input  bit0=0  base0=LSB of Input  dbl_ovrd=off  block_type=slice
  slice3 : xbsIndex_r4/Slice  nbits=1  boolean_output=on  mode=Upper Bit Location + Width  bit1=-1  base1=MSB of Input  bit0=0  base0=LSB of Input  dbl_ovrd=off  block_type=slice
  slice4 : xbsIndex_r4/Slice  nbits=1  boolean_output=on  mode=Upper Bit Location + Width  bit1=0  base1=MSB of Input  bit0=0  base0=LSB of Input  dbl_ovrd=off  block_type=slice
  msb_out4 : Outport
  out3 : Outport  Port=2
  out2 : Outport  Port=3
  lsb_out1 : Outport  Port=4
  wires:
  bus_in/1 -> slice4/1, slice3/1, slice2/1, slice1/1
  slice4/1 -> msb_out4/1
  slice3/1 -> out3/1
  slice2/1 -> out2/1
  slice1/1 -> lsb_out1/1
